simulink model "hopper_6dof"  (R2026b)
settings: Solver=FixedStepAuto  StopTime=tgrid(end)  FixedStep=1e-3  RelTol=1e-5
undefined symbols (not defined in the file): cg_init, controller_start_time, fdir_params, fsw_latency, fsw_period, g, IN, K1flat, K1flat_lo, K2grid, Klqi, nav_dt, nav_g, nav_init, nav_Qc, nav_reset, OUT, p, sensor_params, Target_Trajectory, tgrid, u_hold_command, unom, VEH
libraries: fl_lib x43, nesl_utility x31, SimscapeFluids_lib x13, slpidlib x3, simulink_extras x2, commrandsrc3 x1, dspsrcs4 x1, matrix_library x1, aerolibutil x1
(part 5 of 6)

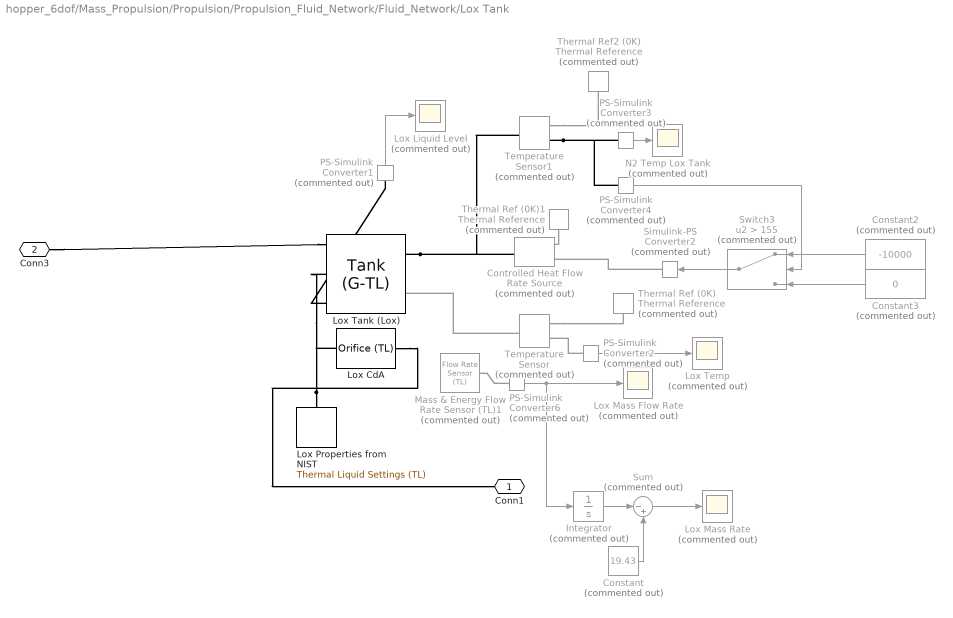
== system hopper_6dof/Mass_Propulsion/Propulsion/Propulsion_Fluid_Network/Fluid_Network/Lox Tank ==
  Constant : Constant  Commented=on  Value=19.43
  Constant2 : Constant  Commented=on  Value=-10000
  Constant3 : Constant  Commented=on  Value=0
  Controlled Heat Flow Rate Source : fl_lib/Thermal/Thermal Sources/Controlled Heat Flow Rate Source  Commented=on
  Integrator : Integrator  Commented=on
  Lox CdA : SimscapeFluids_lib/Thermal Liquid/Valves & Orifices/Orifice (TL)  orifice_type=foundation.enum.constant_variable.constant  constant_orifice_spec=fluids.thermal_liquid.valves.enum.ConstantOrificeSpec.Area  variable_orifice_spec=fluids.thermal_liquid.valves.enum.orifice_spec.linear  orifice_area_constant=100 mm^2  p_diff_TLU_constant=[-4, -3, -2, -1, -.5, 0, .5, 1, 2, 3, 4] MPa  vol_flow_TLU_constant=[-2.44, -2.12, -1.68, -1.22, -.84, 0, .85, 1.21, 1.7, 2.09, 2.41] .* 1e-3 m^3/s  mdot_TLU_constant=[-2.44, -2.12, -1.68, -1.22, -.84, 0, .85, 1.21, 1.7, 2.09, 2.41] kg/s  S_min=0 m  del_S=5e-3 m  open_orientation=fluids.thermal_liquid.valves.enum.orifice_orientation.positive  area_max=1e-4 m^2  area_leak=1e-10 m^2  S_TLU=[0, .002, .004, .007, .017] m  orifice_area_TLU=[1e-09, 2.0352e-07, 4.0736e-05, .00011438, .00034356] m^2  Cd=1  Re_c=150  smoothing_factor=0.01  pressure_recovery=simscape.enum.onoff.off  S_flow_TLU=[0, .002, .004, .007, .017] m  p_diff_TLU=[.3, .5, .7] MPa  vol_flow_TLU=1e-3 * [1.7e-05, 2e-05, 2.6e-05; .0035, .0045, .0053; .7, .9, 1.06; 1.96, 2.5, 3; 6, 7.7, 9.13] m^3/s  mdot_TLU=[1.7e-05, 2e-05, 2.6e-05; .0035, .0045, .0053; .7, .9, 1.06; 1.96, 2.5, 3; 6, 7.7, 9.13] kg/s  T_ref_in=293.15 K  p_ref_in=0.101325 MPa  area=0.01 m^2
  Lox Liquid Level : Scope  Commented=on
      settings: ActiveDisplayYMinimum=0.2716109686745361  ActiveDisplayYMaximum=0.57353060563413627  DataLoggingVariableName=ScopeData8
  Lox Mass Flow Rate : Scope  Commented=on
      settings: ActiveDisplayYMinimum=-0.047859120665806151  ActiveDisplayYMaximum=0.43156982443661435  DataLoggingVariableName=ScopeData9
  Lox Mass Rate : Scope  Commented=on
      settings: ActiveDisplayYMinimum=1.5375974928550786  ActiveDisplayYMaximum=10.60693361190499  DataLoggingVariableName=ScopeData19
  Lox Properties from NIST : fl_lib/Thermal Liquid/Utilities/Thermal Liquid Settings (TL)  table_dimensions=foundation.enum.table_dimensions_TL.two_dimensional  T_TLU=[70 : 10 : 130]' K  p_TLU=[10:10:600] psi  T_atm=100 K  p_atm=0.101325 MPa  pT_region_flag=foundation.enum.pT_region_TL.min_max  T_min=70 K  T_max=130 K  p_min=10 psi  p_max=600 psi  T_min_1D=273.16 K  T_max_1D=363.16 K  p_min_1D=0.05 MPa  p_max_1D=50 MPa  pT_validity_TLU=[1, 1, 1, 1, 1, 1, 1, 1, 1, 1, 1, 1; 1, 1, 1, 1, 1, 1, 1, 1, 1, 1, 1, 1; 1, 1, 1, 1, 1, 1, 1, 1, 1, 1, 1, 1; 1, 1, 1, 1, 1, 1, 1, 1, 1, 1, 1, 1; 1, 1, 1, 1, 1, 1, 1, 1, 1, 1, 1, 1; 0, 1, 1, 1, 1, 1, 1, 1, 1, 1, 1, 1; 0, 1, 1, 1, 1, 1, 1, 1, 1, 1, 1, 1; 0, 1, 1, 1, 1, 1, 1, 1, 1, 1, 1, 1; 0, 1, 1, 1, 1, 1, 1, 1, 1, 1, 1, 1; 0, 1, 1, 1, 1, 1, 1, 1, 1, 1, 1, 1; 0, 0, 1, 1, 1, 1, 1, 1, 1, 1, 1, 1]  properties_range_check=simscape.enum.assert.action.error  rho_parameterization_2D=foundation.enum.rho_parameterization_2D.rho_table  rho_parameterization_1D=foundation.enum.rho_parameterization_1D.rho_vector  rho_TLU=[1237,1190.5,1142.1,1141,1141,1141,1141] kg/m^3  beta_TLU=[1.9649, 1.9654, 1.9929, 2.0213, 2.0499, 2.0787, 2.1078, 2.1372, 2.1668, 2.1966, 2.2268, 2.2572; 2.0913, 2.0918, 2.1191, 2.1471, 2.1752, 2.2036, 2.2322, 2.261, 2.2899, 2.3191, 2.3485, 2.3781; 2.1786, 2.1791, 2.2067, 2.235, 2.2634, 2.2919, 2.3206, 2.3494, 2.3784, 2.4075, 2.4367, 2.4661; 2.2332, 2.2337, 2.2619, 2.2908, 2.3197, 2.3487, 2.3778, 2.407, 2.4363, 2.4657, 2.4951, 2.5246; 2.26, 2.2605, 2.2895, 2.3191, 2.3487, 2.3784, 2.4081, 2.4378, 2.4675, 2.4973, 2.5272, 2.5571; 2.2638, 2.2638, 2.2936, 2.324, 2.3544, 2.3848, 2.4151, 2.4455, 2.4758, 2.5062, 2.5365, 2.5669; 2.2472, 2.2472, 2.2779, 2.3092, 2.3403, 2.3715, 2.4025, 2.4336, 2.4646, 2.4955, 2.5264, 2.5573; 2.214, 2.214, 2.2455, 2.2776, 2.3096, 2.3415, 2.3733, 2.405, 2.4367, 2.4683, 2.4998, 2.5313; 2.1668, 2.1668, 2.1992, 2.2321, 2.2649, 2.2976, 2.3301, 2.3626, 2.3949, 2.4272, 2.4593, 2.4914; 2.1081, 2.1081, 2.1413, 2.175, 2.2086, 2.2421, 2.2754, 2.3085, 2.3415, 2.3744, 2.4072, 2.4399; 2.0494, 2.0494, 2.0739, 2.1084, 2.1428, 2.177, 2.211, 2.2449, 2.2786, 2.3121, 2.3455, 2.3788] GPa  alpha_TLU=1e-4 * [-.679, -.676, -.49, -.307, -.13, .041, .206, .365, .519, .668, .811, .949; .878, .881, .998, 1.114, 1.227, 1.337, 1.445, 1.549, 1.651, 1.75, 1.846, 1.939; 2.068, 2.069, 2.141, 2.213, 2.283, 2.352, 2.42, 2.486, 2.551, 2.614, 2.676, 2.736; 3.034, 3.035, 3.074, 3.113, 3.152, 3.191, 3.229, 3.267, 3.305, 3.341, 3.377, 3.413; 3.855, 3.856, 3.87, 3.884, 3.899, 3.914, 3.93, 3.946, 3.961, 3.977, 3.993, 4.009; 4.578, 4.578, 4.572, 4.566, 4.562, 4.558, 4.555, 4.552, 4.55, 4.549, 4.548, 4.547; 5.233, 5.233, 5.209, 5.186, 5.165, 5.144, 5.125, 5.107, 5.09, 5.074, 5.059, 5.045; 5.84, 5.84, 5.801, 5.762, 5.725, 5.691, 5.657, 5.625, 5.595, 5.566, 5.538, 5.512; 6.414, 6.414, 6.36, 6.307, 6.256, 6.208, 6.161, 6.117, 6.074, 6.033, 5.994, 5.956; 6.967, 6.967, 6.898, 6.831, 6.766, 6.705, 6.646, 6.589, 6.535, 6.482, 6.432, 6.384; 7.519, 7.519, 7.423, 7.342, 7.264, 7.189, 7.118, 7.049, 6.983, 6.92, 6.859, 6.8] 1/K  rho_TLU_2=|  rho_ref_3=998.21 kg/m^3  T_ref_3=293.16 K  p_ref_3=0.101325 MPa  beta_const_3=2.1791 GPa  alpha_const_3=2.0691e-4 1/K  rho_TLU_4=[999.84; 999.7; 998.2; 995.65; 992.21; 988.03; 983.19; 977.76; 971.78; 965.3; 958.8] kg/m^3  beta_const_4=2.1791 GPa  p_ref_4=0.101325 MPa  rho_ref_5=998.21 kg/m^3  T_ref_5=293.16 K  p_ref_5=0.101325 MPa  beta_const_5=2.1791 GPa  alpha_const_5=2.0691e-4 1/K  u_parameterization_2D=foundation.enum.u_parameterization_2D.u_cp  u_parameterization_1D=foundation.enum.u_parameterization_1D.u  u_TLU=|  cp_TLU=|  u_TLU_2=[.0002, .0018, .086, .1588, .219, .267, .3034, .3288, .3436, .3483, .3435, .3294; 42.062, 42.06, 41.935, 41.804, 41.668, 41.527, 41.382, 41.233, 41.081, 40.924, 40.763, 40.599; 83.953, 83.948, 83.651, 83.349, 83.049, 82.749, 82.451, 82.153, 81.856, 81.56, 81.265, 80.971; 125.77, 125.76, 125.31, 124.86, 124.41, 123.97, 123.53, 123.1, 122.68, 122.25, 121.84, 121.42; 167.57, 167.56, 166.96, 166.37, 165.79, 165.21, 164.65, 164.09, 163.54, 163, 162.46, 161.94; 209.36, 209.36, 208.63, 207.9, 207.19, 206.48, 205.79, 205.11, 204.45, 203.79, 203.14, 202.5; 251.19, 251.19, 250.33, 249.47, 248.62, 247.79, 246.98, 246.18, 245.39, 244.62, 243.86, 243.12; 293.06, 293.06, 292.07, 291.07, 290.1, 289.14, 288.2, 287.28, 286.38, 285.49, 284.62, 283.77; 334.99, 334.99, 333.86, 332.73, 331.63, 330.54, 329.48, 328.44, 327.41, 326.41, 325.43, 324.46; 377, 377, 375.73, 374.46, 373.22, 372, 370.81, 369.64, 368.5, 367.38, 366.27, 365.19; 419.01, 419.01, 417.69, 416.27, 414.89, 413.54, 412.21, 410.91, 409.64, 408.4, 407.17, 405.98] kJ/kg  cp_TLU_3=[4.2199, 4.2194, 4.1957, 4.1726, 4.1508, 4.13, 4.1103, 4.0916, 4.0738, 4.0569, 4.0408, 4.0254; 4.1955, 4.1951, 4.1769, 4.1592, 4.1422, 4.1259, 4.1103, 4.0954, 4.0812, 4.0676, 4.0545, 4.0421; 4.1843, 4.184, 4.169, 4.1543, 4.1401, 4.1264, 4.1133, 4.1007, 4.0885, 4.0768, 4.0656, 4.0548; 4.1801, 4.1798, 4.1667, 4.1538, 4.1413, 4.1293, 4.1177, 4.1064, 4.0956, 4.0851, 4.075, 4.0653; 4.1796, 4.1794, 4.1675, 4.1558, 4.1444, 4.1334, 4.1227, 4.1123, 4.1023, 4.0926, 4.0832, 4.0741; 4.1813, 4.1813, 4.1702, 4.1592, 4.1484, 4.138, 4.1279, 4.1181, 4.1086, 4.0993, 4.0903, 4.0816; 4.185, 4.185, 4.1742, 4.1636, 4.1532, 4.1432, 4.1334, 4.1239, 4.1146, 4.1056, 4.0969, 4.0884; 4.1901, 4.1901, 4.1795, 4.169, 4.1588, 4.1489, 4.1393, 4.1299, 4.1207, 4.1118, 4.1032, 4.0947; 4.1968, 4.1968, 4.1862, 4.1757, 4.1655, 4.1555, 4.1458, 4.1364, 4.1273, 4.1183, 4.1096, 4.1012; 4.2052, 4.2052, 4.1944, 4.1837, 4.1733, 4.1632, 4.1534, 4.1438, 4.1345, 4.1255, 4.1166, 4.108; 4.2136, 4.2136, 4.2045, 4.1935, 4.1828, 4.1724, 4.1623, 4.1524, 4.1429, 4.1335, 4.1245, 4.1157] kJ/(K*kg)  u_TLU_4=[.0018; 42.06; 83.948; 125.76; 167.56; 209.36; 251.19; 293.06; 334.99; 377; 418.01] kJ/kg  cp_TLU_5=[4.2199; 4.1955; 4.1843; 4.1801; 4.1796; 4.1813; 4.185; 4.1901; 4.1968; 4.2052; 4.2136] kJ/(K*kg)  nu_TLU=|  nu_TLU_2=[1.7917; 1.3061; 1.0032; .8006; .6577; .553; .4739; .4127; .3643; .3254; .2866] mm^2/s  k_TLU=|  k_TLU_2=[561.04; 580.02; 598.44; 615.48; 630.6; 643.61; 654.39; 663.13; 670.02; 675.27; 680.52] mW/(K*m)  air_fraction=0  R_air=0.287 kJ/(K*kg)  air_dissolution_model=false  p_crit=3 MPa
      rho_TLU_2=|
      | [1237.088,1237.184,1237.28,1237.376,1237.504,1237.6,1237.696,1237.792,1237.888,1237.984,1238.08,1238.176,1238.272,1238.4,1238.496,1238.592,1238.688,1238.784,1238.88,1238.976,1239.072,1239.168,1239.264,1239.392,1239.488,1239.584,1239.68,1239.776,1239.872,1239.968,1240.064,1240.16,1240.256,1240.352,1240.448,1240.544,1240.64,1240.768,1240.864,1240.96,1241.056,1241.152,1241.248,1241.344,1241.44,1241.536,1241.632,1241.728,1241.824,1241.92,1242.0,1242.1,1242.2,1242.3,1242.4,1242.5,1242.6,1242.7,1242.71,1242.8;
      | 
      | 1190.56,1190.688,1190.816,1190.944,1191.072,1191.2,1191.296,1191.424,1191.552,1191.68,1191.808,1191.904,1192.032,1192.16,1192.288,1192.416,1192.512,1192.64,1192.768,1192.896,1192.992,1193.12,1193.248,1193.376,1193.504,1193.6,1193.728,1193.856,1193.984,1194.08,1194.208,1194.336,1194.464,1194.56,1194.688,1194.816,1194.912,1195.04,1195.168,1195.296,1195.392,1195.52,1195.648,1195.744,1195.872,1196,1196.128,1196.224,1196.352,1196.48,1196.5,1196.7,1196.8,1196.9,1197.0,1197.1,1197.2,1197.4,1197.5,1197.6;
      | 
      | 3.013,1142.24,1142.4,1142.528,1142.688,1142.848,1143.008,1143.136,1143.296,1143.456,1143.616,1143.744,1143.904,1144.064,1144.224,1144.352,1144.512,1144.672,1144.832,1144.96,1145.12,1145.28,1145.408,1145.568,1145.728,1145.856,1146.016,1146.176,1146.304,1146.464,1146.624,1146.752,1146.912,1147.072,1147.2,1147.36,1147.488,1147.648,1147.808,1147.936,1148.096,1148.256,1148.384,1148.544,1148.672,1148.832,1148.96,1149.12,1149.28,1149.408,1149.5,1149.7,1149.8,1150.0,1150.1,1150.2,1150.4,1150.5,1150.7,1150.8;
      | 
      | 2.697,5.487,8.38,1090.976,1091.2,1091.392,1091.584,1091.776,1091.968,1092.16,1092.384,1092.576,1092.768,1092.96,1093.152,1093.344,1093.536,1093.728,1093.92,1094.112,1094.304,1094.496,1094.688,1094.88,1095.072,1095.264,1095.456,1095.648,1095.84,1096.032,1096.224,1096.416,1096.608,1096.8,1096.992,1097.184,1097.376,1097.536,1097.728,1097.92,1098.112,1098.304,1098.496,1098.688,1098.848,1099.04,1099.232,1099.424,1099.616,1099.776,1099.9,1100.1,1100.3,1100.5,1100.7,1100.9,1101.0,1101.2,1101.4,1101.6;
      | 
      | 2.442,4.948,7.521,10.167,12.894,15.709,18.623,1035.552,1035.808,1036.064,1036.352,1036.608,1036.864,1037.12,1037.408,1037.664,1037.92,1038.176,1038.432,1038.688,1038.944,1039.2,1039.488,1039.744,1040,1040.256,1040.512,1040.768,1041.024,1041.248,1041.504,1041.76,1042.016,1042.272,1042.528,1042.784,1043.04,1043.264,1043.52,1043.776,1044.032,1044.256,1044.512,1044.768,1045.024,1045.248,1045.504,1045.76,1045.984,1046.24,1046.4,1046.7,1046.9,1047.2,1047.4,1047.6,1047.9,1048.1,1048.4,1048.6;
      | 
      | 2.233,4.51,6.834,9.207,11.634,14.116,16.659,19.267,21.944,24.697,27.532,30.458,33.485,36.621,973.952,974.336,974.72,975.104,975.488,975.84,976.224,976.608,976.96,977.344,977.728,978.08,978.464,978.816,979.168,979.552,979.904,980.256,980.64,980.992,981.344,981.696,982.048,982.4,982.752,983.104,983.456,983.808,984.16,984.512,984.864,985.216,985.536,985.888,986.24,986.56,986.87,987.21,987.55,987.89,988.22,988.56,988.89,989.22,989.55,989.88;
      | 
      | 2.057,4.146,6.268,8.426,10.62,12.852,15.125,17.441,19.801,22.209,24.666,27.176,29.743,32.368,35.059,37.818,40.653,43.565,46.563,49.658,52.858,56.17,59.61,63.197,66.944,902.912,903.52,904.128,904.704,905.312,905.92,906.496,907.104,907.68,908.256,908.832,909.408,909.952,910.528,911.104,911.648,912.224,912.768,913.312,913.856,914.4,914.944,915.488,916,916.544,917.03,917.56,918.08,918.6,919.12,919.63,920.14,920.65,921.16,921.66] kg/m^3
      u_TLU=|
      | [-167.43125,-167.44375,-167.459375,-167.475,-167.4875,-167.503125,-167.515625,-167.53125,-167.546875,-167.559375,-167.575,-167.5875,-167.603125,-167.615625,-167.63125,-167.646875,-167.659375,-167.675,-167.6875,-167.703125,-167.715625,-167.73125,-167.74375,-167.759375,-167.771875,-167.7875,-167.8,-167.815625,-167.828125,-167.84375,-167.85625,-167.871875,-167.884375,-167.9,-167.9125,-167.928125,-167.940625,-167.95625,-167.96875,-167.984375,-167.996875,-168.0125,-168.025,-168.040625,-168.053125,-168.06875,-168.08125,-168.09375,-168.109375,-168.121875,-168.14,-168.16,-168.17,-168.18,-168.20,-168.21,-168.23,-168.24,-168.25,-168.27;
      | -150.64375,-150.6625,-150.68125,-150.696875,-150.715625,-150.734375,-150.753125,-150.771875,-150.790625,-150.809375,-150.825,-150.84375,-150.8625,-150.88125,-150.9,-150.91875,-150.934375,-150.953125,-150.971875,-150.990625,-151.00625,-151.025,-151.04375,-151.0625,-151.078125,-151.096875,-151.115625,-151.134375,-151.15,-151.16875,-151.1875,-151.20625,-151.221875,-151.240625,-151.259375,-151.275,-151.29375,-151.3125,-151.328125,-151.346875,-151.365625,-151.38125,-151.4,-151.41875,-151.434375,-151.453125,-151.46875,-151.4875,-151.50625,-151.521875,-151.55,-151.56,-151.58,-151.60,-151.62,-151.63,-151.65,-151.67,-151.68,-151.70;
      | 57.3375,-133.784375,-133.80625,-133.83125,-133.853125,-133.878125,-133.9,-133.925,-133.946875,-133.971875,-133.99375,-134.01875,-134.040625,-134.065625,-134.0875,-134.1125,-134.134375,-134.159375,-134.18125,-134.203125,-134.228125,-134.25,-134.271875,-134.296875,-134.31875,-134.34375,-134.365625,-134.3875,-134.4125,-134.434375,-134.45625,-134.478125,-134.503125,-134.525,-134.546875,-134.56875,-134.59375,-134.615625,-134.6375,-134.659375,-134.684375,-134.70625,-134.728125,-134.75,-134.771875,-134.79375,-134.81875,-134.840625,-134.8625,-134.884375,-134.91,-134.93,-134.96,-134.98,-135.00,-135.02,-135.04,-135.07,-135.09,-135.11;
      | 63.946875,63.184375,62.378125,-116.6875,-116.71875,-116.75,-116.78125,-116.8125,-116.84375,-116.871875,-116.903125,-116.934375,-116.965625,-116.996875,-117.025,-117.05625,-117.0875,-117.11875,-117.146875,-117.178125,-117.209375,-117.2375,-117.26875,-117.296875,-117.328125,-117.359375,-117.3875,-117.41875,-117.446875,-117.478125,-117.50625,-117.5375,-117.565625,-117.596875,-117.625,-117.653125,-117.684375,-117.7125,-117.74375,-117.771875,-117.8,-117.83125,-117.859375,-117.8875,-117.915625,-117.946875,-117.975,-118.003125,-118.03125,-118.0625,-118.09,-118.12,-118.15,-118.18,-118.21,-118.24,-118.27,-118.29,-118.32,-118.35;
      | 70.5375,69.884375,69.209375,68.515625,67.796875,67.046875,66.25625,-99.165625,-99.209375,-99.25,-99.29375,-99.334375,-99.375,-99.415625,-99.459375,-99.5,-99.540625,-99.58125,-99.621875,-99.6625,-99.703125,-99.74375,-99.784375,-99.825,-99.865625,-99.90625,-99.946875,-99.9875,-100.028125,-100.065625,-100.10625,-100.146875,-100.184375,-100.225,-100.265625,-100.303125,-100.34375,-100.38125,-100.421875,-100.459375,-100.5,-100.5375,-100.578125,-100.615625,-100.653125,-100.69375,-100.73125,-100.76875,-100.809375,-100.846875,-100.89,-100.93,-110.96,-101.00,-101.04,-101.08,-101.11,-101.15,-101.19,-101.23;
      | 77.11875,76.55625,75.978125,75.390625,74.7875,74.16875,73.5375,72.8875,72.215625,71.525,70.809375,70.0625,69.28125,68.459375,-80.9625,-81.021875,-81.08125,-81.140625,-81.2,-81.25625,-81.315625,-81.375,-81.43125,-81.490625,-81.546875,-81.60625,-81.6625,-81.71875,-81.778125,-81.834375,-81.890625,-81.946875,-82.003125,-82.059375,-82.115625,-82.16875,-82.225,-82.28125,-82.334375,-82.390625,-82.446875,-82.5,-82.553125,-82.609375,-82.6625,-82.715625,-82.76875,-82.821875,-82.878125,-82.93125,-82.986,-83.039,-83.091,-83.144,-83.196,-83.248,-83.300,-83.352,-83.404,-83.455;
      | 83.6875,83.2,82.7,82.19375,81.68125,81.15625,80.621875,80.078125,79.525,78.959375,78.38125,77.790625,77.1875,76.56875,75.9375,75.284375,74.6125,73.921875,73.209375,72.46875,71.7,70.896875,70.05625,69.175,68.240625,-61.65625,-61.75,-61.840625,-61.934375,-62.025,-62.115625,-62.203125,-62.29375,-62.38125,-62.471875,-62.559375,-62.646875,-62.73125,-62.81875,-62.903125,-62.9875,-63.075,-63.159375,-63.240625,-63.325,-63.40625,-63.490625,-63.571875,-63.653125,-63.734375,-63.818,-63.898,-63.978,-64.057,-64.136,-64.215,-64.293,-64.371,-64.449,-64.526] kJ/kg
      cp_TLU=|
      | [1.67790625,1.67775,1.67759375,1.67746875,1.6773125,1.67715625,1.677,1.676875,1.67671875,1.6765625,1.6764375,1.67628125,1.67615625,1.676,1.67584375,1.67571875,1.6755625,1.6754375,1.67528125,1.675125,1.675,1.67484375,1.67471875,1.6745625,1.6744375,1.67428125,1.67415625,1.674,1.673875,1.67371875,1.67359375,1.6734375,1.6733125,1.67315625,1.67303125,1.67290625,1.67275,1.672625,1.67246875,1.67234375,1.67221875,1.6720625,1.6719375,1.6718125,1.67165625,1.67153125,1.67140625,1.67125,1.671125,1.671,1.6709,1.6708,1.6707,1.6705,1.6704,1.6703,1.6701,1.67,1.6699,1.6697;
      | 1.681375,1.68115625,1.6809375,1.68071875,1.6805,1.68028125,1.6800625,1.67984375,1.679625,1.67940625,1.6791875,1.67896875,1.67875,1.6785625,1.67834375,1.678125,1.67790625,1.6776875,1.67746875,1.67728125,1.6770625,1.67684375,1.676625,1.6764375,1.67621875,1.676,1.67578125,1.67559375,1.675375,1.6751875,1.67496875,1.67475,1.6745625,1.67434375,1.67415625,1.6739375,1.67375,1.67353125,1.67334375,1.673125,1.6729375,1.67271875,1.67253125,1.6723125,1.672125,1.6719375,1.67171875,1.67153125,1.6713125,1.671125,1.671,1.6708,1.6706,1.6704,1.6702,1.67,1.6698,1.6696,1.6694,1.6692;
      | 0.93946875,1.69859375,1.69825,1.697875,1.69753125,1.6971875,1.69684375,1.69646875,1.696125,1.69578125,1.6954375,1.69509375,1.69475,1.69440625,1.6940625,1.69371875,1.693375,1.69303125,1.69271875,1.692375,1.69203125,1.6916875,1.691375,1.69103125,1.6906875,1.690375,1.69003125,1.68971875,1.689375,1.6890625,1.68871875,1.68840625,1.6880625,1.68775,1.6874375,1.68709375,1.68678125,1.68646875,1.68615625,1.68584375,1.6855,1.6851875,1.684875,1.6845625,1.68425,1.6839375,1.683625,1.6833125,1.683,1.6826875,1.6825,1.6821,1.6818,1.6815,1.6812,1.6809,1.6806,1.6803,1.68,1.6797;
      | 0.92621875,0.947625,0.97703125,1.73728125,1.7366875,1.73609375,1.73553125,1.7349375,1.734375,1.73378125,1.73321875,1.73265625,1.73209375,1.7315,1.7309375,1.730375,1.72984375,1.72928125,1.72871875,1.72815625,1.727625,1.7270625,1.72653125,1.72596875,1.7254375,1.724875,1.72434375,1.7238125,1.72328125,1.72275,1.72221875,1.7216875,1.72115625,1.720625,1.720125,1.71959375,1.7190625,1.7185625,1.71803125,1.71753125,1.71703125,1.7165,1.716,1.7155,1.715,1.7145,1.714,1.7135,1.713,1.7125,1.7121,1.7116,1.7111,1.7106,1.7101,1.7096,1.7092,1.7087,1.7082,1.7077;
      | 0.9244375,0.94053125,0.95809375,0.9775625,0.99996875,1.027,1.06146875,1.806625,1.80559375,1.8045625,1.8035625,1.80253125,1.80153125,1.80053125,1.79953125,1.79853125,1.7975625,1.7965625,1.79559375,1.794625,1.79365625,1.7926875,1.79175,1.79078125,1.78984375,1.78890625,1.78796875,1.78703125,1.786125,1.7851875,1.78428125,1.783375,1.78246875,1.7815625,1.78065625,1.77978125,1.778875,1.778,1.777125,1.77625,1.775375,1.7745,1.77365625,1.77278125,1.7719375,1.77109375,1.77025,1.76940625,1.7685625,1.76771875,1.767,1.7661,1.7653,1.7645,1.7637,1.7629,1.7621,1.7613,1.7605,1.7597;
      | 0.922125,0.93528125,0.9491875,0.96396875,0.97971875,0.9965625,1.01475,1.03465625,1.05665625,1.081375,1.10965625,1.14259375,1.18165625,1.2289375,1.92671875,1.9246875,1.9226875,1.9206875,1.91871875,1.91675,1.9148125,1.912875,1.91096875,1.9090625,1.9071875,1.9053125,1.90346875,1.901625,1.8998125,1.898,1.89621875,1.8944375,1.8926875,1.8909375,1.8891875,1.88746875,1.88575,1.8840625,1.882375,1.88071875,1.8790625,1.87740625,1.87578125,1.87415625,1.87253125,1.8709375,1.869375,1.86778125,1.86621875,1.8646875,1.8632,1.8617,1.8602,1.8587,1.8572,1.8557,1.8542,1.8527,1.8513,1.8498;
      | 0.919875,0.9304375,0.9415,0.95309375,0.96521875,0.9779375,0.99128125,1.00534375,1.0201875,1.03590625,1.0525625,1.070375,1.0894375,1.10996875,1.1321875,1.156375,1.1829375,1.21228125,1.2449375,1.281625,1.32321875,1.370875,1.4260625,1.49084375,1.5679375,2.15015625,2.14528125,2.1404375,2.13571875,2.13103125,2.1264375,2.12190625,2.1174375,2.11303125,2.1086875,2.10440625,2.10015625,2.096,2.09190625,2.08784375,2.08384375,2.07990625,2.07603125,2.0721875,2.06840625,2.06465625,2.06096875,2.0573125,2.05371875,2.05015625,2.0467,2.0433,2.0398,2.0365,2.0331,2.0298,2.0265,2.0233,2.0201,2.017] kJ/(K*kg)
      nu_TLU=|
      | [0.300698091000802,0.300852581346024,0.301007047717574,0.30116149012103,0.301308116983864,0.301462508080155,0.301616875226227,0.301771218427652,0.301925537690001,0.302079833018844,0.302234104419747,0.302388351898276,0.302542575459996,0.302688953488372,0.302843125855877,0.302997274324394,0.303151398899481,0.303305499586691,0.303459576391579,0.303613629319696,0.303767658376592,0.303921663567813,0.304075644898908,0.304221747437453,0.304375677699179,0.304529584118543,0.304683466701084,0.30483732545234,0.304991160377845,0.305144971483135,0.305298758773741,0.305452522255193,0.30560626193302,0.30575997781275,0.305913669899907,0.306067338200015,0.306220982718597,0.306366701913653,0.306528354436908,0.306681923671996,0.306835469148854,0.306988990872995,0.307142488849932,0.307295963085172,0.307449413584225,0.307602840352595,0.307756243395789,0.307909622719307,0.308062978328652,0.308216310229322,0.3083,0.3084,0.3086,0.3088,0.3089,0.3091,0.3093,0.3094,0.3096,0.3098;
      | 0.219484948259643,0.21960412803354,0.219714884583345,0.219834014025848,0.219944722065501,0.220063801208865,0.220188769205974,0.220299406424581,0.220418412289183,0.220529001074114,0.220647956717861,0.220764423980455,0.220883331991088,0.221002214467857,0.221112684183687,0.221231516517725,0.221347877421779,0.221466662194795,0.221585421473413,0.221695772305381,0.221820431318902,0.221930736221,0.222049397945775,0.222159654626874,0.2222782663485,0.222402815013405,0.222513001286725,0.222631540152246,0.222741678280446,0.222866139622136,0.222976231946194,0.223094673525708,0.223213089720578,0.223329091883204,0.223447460759629,0.223557434784938,0.223681743927586,0.22379167224528,0.22390994404134,0.224028190506787,0.224144046471785,0.224262245717345,0.224372055989723,0.224496213236278,0.224614339996254,0.224724080267559,0.224842157361085,0.224957867422824,0.225075897394747,0.225185544263172,0.2253,0.2254,0.2255,0.2256,0.2257,0.2258,0.2259,0.2260,0.2261,0.2262;
      | 2.3012413456229,0.171347527664939,0.171446078431373,0.171540653708268,0.171639152594584,0.171737623900991,0.171836067639072,0.171930548946057,0.1720289408867,0.172127305292027,0.172216897979741,0.172320029656986,0.172418314823622,0.172507831729693,0.172606063148474,0.172709096501776,0.172798537717385,0.172896690056191,0.17299481495975,0.173089016210173,0.173187089562666,0.173285135512713,0.173379267474996,0.173477261934691,0.17357522902469,0.173669291778374,0.17376720743864,0.173865095761907,0.173959089386411,0.174056926340469,0.174146014735432,0.174248660564795,0.174346418905723,0.174435432126318,0.174538005578801,0.174635685399526,0.174729496081876,0.174827124693286,0.174916013828097,0.175018467928526,0.175116018172696,0.175204832371875,0.175307214311589,0.175404686281065,0.17549831457544,0.175595735494833,0.175689319036346,0.175786688944584,0.175884031741612,0.175977546702302,0.1761,0.1762,0.1763,0.1764,0.1765,0.1766,0.1767,0.1768,0.1769,0.1770;
      | 2.85843745179701,1.40626822582527,0.921651836859391,0.139865588243921,0.139956011730205,0.140041341699408,0.140126641651032,0.140221070988921,0.140306309342398,0.14039151772634,0.140481735360459,0.140566880473303,0.140651995666052,0.140737080954472,0.140831284212991,0.140916308133579,0.141001302197641,0.14109540946195,0.141180342255375,0.141265245239975,0.141350118431441,0.141444098470894,0.141528910520623,0.141613692824784,0.141698445399024,0.141783168258977,0.141876990038851,0.141961651917404,0.14204628412907,0.14213088668944,0.142215459614093,0.142309123544348,0.142393635647378,0.142478118161926,0.142562571103527,0.142646994487707,0.14273138832998,0.142819916613214,0.142913362873134,0.142997668318275,0.14308194428255,0.143166190781423,0.143250407830343,0.143334595444749,0.143422930195987,0.143507060707527,0.143600259089983,0.14368432924877,0.143768370049181,0.143856567155493,0.1439,0.1440,0.1441,0.1442,0.1443,0.1444,0.1445,0.1446,0.1447,0.1448;
      | 3.46737713402251,1.71372728154712,1.12873888439774,0.836008560727662,0.660077242834098,0.542540026888291,0.458327247577153,0.117367355767745,0.117454200006179,0.117541001328103,0.117624127709504,0.117710841513861,0.117797512499228,0.11787449861154,0.117957447792961,0.118043991118512,0.118130491752736,0.118216949727214,0.118303365073495,0.1183897378231,0.118476068007515,0.118562355658199,0.118635328161556,0.118721531453896,0.118807692307692,0.118893810754276,0.118979886824948,0.119065920550978,0.119142306037133,0.119231921693967,0.11931783267275,0.119403701428352,0.119479931210269,0.119565717969973,0.119651462598606,0.119727575413508,0.119813238226722,0.119902536654193,0.119978534191966,0.120064075050586,0.120149573959419,0.120229139214905,0.120314558377501,0.1203999356795,0.120475701993447,0.1205646889542,0.120640380142018,0.120725596695226,0.120814467525316,0.120890044349289,0.1209,0.1210,0.1211,0.1212,0.1213,0.1214,0.1215,0.1216,0.1217,0.1218;
      | 4.1267001805882,2.04580731568864,1.35196675251698,1.00487235854303,0.7964258698941,0.657316838191957,0.557841913177103,0.483103647295255,0.424857092860476,0.378142856217365,0.33980229895745,0.307732767043843,0.280461582568807,0.256971447920308,0.10005421211723,0.100145124474514,0.100234939264609,0.100324683315831,0.100414356711718,0.100506230529595,0.100595764906415,0.100684204921524,0.100775876187357,0.100863155654509,0.100950366564116,0.101041837068542,0.101127890244301,0.101218206486204,0.101308457792738,0.101394310868642,0.101483410619816,0.101571426239676,0.1016570810899,0.101744968358559,0.101833811589004,0.101925647043484,0.102011306982958,0.102096905537459,0.102182442772948,0.102267918755289,0.102353333550255,0.102438687223523,0.102523979840676,0.102609211467204,0.102694382168502,0.102779492009874,0.102867881031236,0.102952870914343,0.103037800129786,0.103126013623094,0.1032,0.1033,0.1034,0.1035,0.1036,0.1037,0.1038,0.1039,0.1040,0.1041;
      | 4.83498179753255,2.40209651898734,1.59107297835409,1.18538739080896,0.941822099014675,0.779460462105368,0.663319546406584,0.576172412527751,0.508300473504743,0.453967464914556,0.409426000882177,0.372272625579917,0.34075198769191,0.313704893722195,0.29016634720701,0.269557031646641,0.251274204974811,0.234983289261055,0.220367156896433,0.207118346436396,0.19507128586996,0.184049735088019,0.173931715696801,0.164549470859284,0.155831739961759,0.0860150269350723,0.0861198423941916,0.0862234108444822,0.0863298935342388,0.0864320808737761,0.0865341310490993,0.0866379995057893,0.0867375736409497,0.0868400757976379,0.0869413469330233,0.0870424897010669,0.0871424047292304,0.0872452612885075,0.0873438268784705,0.0874422678420905,0.0875425602864263,0.0876385624583436,0.0877386148506521,0.0878363582215059,0.0879339852230548,0.0880314960629921,0.0881288909485171,0.0882239854591212,0.0883231441048035,0.0884180137560226,0.0885,0.0886,0.0887,0.0888,0.0889,0.0890,0.0891,0.0892,0.0893,0.0894] mm^2/s
      k_TLU=|
      | [0.17977,0.1798,0.17984,0.17987,0.17991,0.17994,0.17998,0.18001,0.18005,0.18008,0.18012,0.18015,0.18019,0.18022,0.18026,0.18029,0.18033,0.18037,0.1804,0.18044,0.18047,0.18051,0.18054,0.18058,0.18061,0.18065,0.18068,0.18072,0.18075,0.18079,0.18082,0.18086,0.18089,0.18093,0.18096,0.181,0.18103,0.18107,0.1811,0.18113,0.18117,0.1812,0.18124,0.18127,0.18131,0.18134,0.18138,0.18141,0.18145,0.18148,0.18152,0.18155,0.18159,0.18162,0.18166,0.18169,0.18173,0.18176,0.18179,0.18183;
      | 0.16551,0.16556,0.1656,0.16564,0.16569,0.16573,0.16577,0.16582,0.16586,0.1659,0.16594,0.16599,0.16603,0.16607,0.16612,0.16616,0.1662,0.16624,0.16629,0.16633,0.16637,0.16642,0.16646,0.1665,0.16654,0.16659,0.16663,0.16667,0.16671,0.16676,0.1668,0.16684,0.16688,0.16693,0.16697,0.16701,0.16705,0.1671,0.16714,0.16718,0.16722,0.16727,0.16731,0.16735,0.16739,0.16743,0.16748,0.16752,0.16756,0.1676,0.16764,0.16769,0.16773,0.16777,0.16781,0.16785,0.1679,0.16794,0.16798,0.16802;
      | 0.0080721,0.15115,0.1512,0.15125,0.1513,0.15136,0.15141,0.15146,0.15151,0.15156,0.15162,0.15167,0.15172,0.15177,0.15182,0.15187,0.15193,0.15198,0.15203,0.15208,0.15213,0.15218,0.15223,0.15228,0.15234,0.15239,0.15244,0.15249,0.15254,0.15259,0.15264,0.15269,0.15274,0.1528,0.15285,0.1529,0.15295,0.153,0.15305,0.1531,0.15315,0.1532,0.15325,0.1533,0.15335,0.1534,0.15345,0.15351,0.15356,0.15361,0.15366,0.15371,0.15376,0.15381,0.15386,0.15391,0.15396,0.15401,0.15406,0.15411;
      | 0.0090396,0.0091429,0.0092543,0.13659,0.13665,0.13671,0.13677,0.13684,0.1369,0.13696,0.13702,0.13709,0.13715,0.13721,0.13727,0.13733,0.1374,0.13746,0.13752,0.13758,0.13764,0.13771,0.13777,0.13783,0.13789,0.13795,0.13801,0.13807,0.13814,0.1382,0.13826,0.13832,0.13838,0.13844,0.1385,0.13856,0.13862,0.13868,0.13875,0.13881,0.13887,0.13893,0.13899,0.13905,0.13911,0.13917,0.13923,0.13929,0.13935,0.13941,0.13947,0.13953,0.13959,0.13965,0.13971,0.13977,0.13983,0.13989,0.13995,0.14001;
      | 0.01,0.010091,0.010187,0.010288,0.010395,0.010509,0.010632,0.12192,0.122,0.12208,0.12215,0.12223,0.1223,0.12238,0.12245,0.12253,0.1226,0.12268,0.12275,0.12283,0.1229,0.12298,0.12305,0.12312,0.1232,0.12327,0.12335,0.12342,0.12349,0.12357,0.12364,0.12371,0.12379,0.12386,0.12393,0.12401,0.12408,0.12415,0.12422,0.1243,0.12437,0.12444,0.12451,0.12459,0.12466,0.12473,0.1248,0.12487,0.12495,0.12502,0.12509,0.12516,0.12523,0.1253,0.12537,0.12545,0.12552,0.12559,0.12566,0.12573;
      | 0.010953,0.011035,0.011119,0.011207,0.011299,0.011395,0.011495,0.0116,0.01171,0.011826,0.011949,0.01208,0.012221,0.012373,0.10725,0.10734,0.10743,0.10753,0.10762,0.10771,0.1078,0.1079,0.10799,0.10808,0.10817,0.10826,0.10836,0.10845,0.10854,0.10863,0.10872,0.10881,0.1089,0.10899,0.10908,0.10917,0.10926,0.10935,0.10944,0.10953,0.10962,0.1097,0.10979,0.10988,0.10997,0.11006,0.11015,0.11023,0.11032,0.11041,0.1105,0.11058,0.11067,0.11076,0.11084,0.11093,0.11101,0.1111,0.11119,0.11127;
      | 0.011896,0.01197,0.012047,0.012126,0.012206,0.01229,0.012376,0.012465,0.012557,0.012653,0.012752,0.012855,0.012962,0.013074,0.013192,0.013315,0.013444,0.01358,0.013725,0.013878,0.014043,0.014219,0.01441,0.014619,0.014849,0.092711,0.092831,0.092951,0.09307,0.093189,0.093308,0.093426,0.093544,0.093661,0.093777,0.093894,0.09401,0.094125,0.09424,0.094355,0.094469,0.094583,0.094696,0.094809,0.094922,0.095034,0.095146,0.095257,0.095368,0.095479,0.09559,0.0957,0.095809,0.095919,0.096028,0.096136,0.096245,0.096353,0.09646,0.096568] W/(m*K)
  Lox Tank (Lox) : SimscapeFluids_lib/Thermal Liquid/Tanks & Accumulators/Tank (G-TL)  num_inlet=1  volume_total=19.88 l  volume_spec=fluids.thermal_liquid.tanks_accumulators.enum.TankVolumeSpec.Constant  tank_area=0.35 ft^2  level_TLU=[0, 3, 5] m  volume_TLU=[0, 4, 6] m^3  inlet_areas_A1B1=[1, 1] in^2  inlet_height_A2=0 in  inlet_area_A2=0.78 in^2  inlet_heights_A2B2=[.1, .1] m  inlet_areas_A2B2=[.01, .01] m^2  inlet_heights_A2B2C2=[.1, .1, .1] m  inlet_areas_A2B2C2=[.01, .01, .01] m^2  inlet_heights_A2B2C2D2=0.1 * ones(1, 4) m  inlet_areas_A2B2C2D2=0.01 * ones(1, 4) m^2  inlet_heights_A2B2C2D2E2=0.1 * ones(1, 5) m  inlet_areas_A2B2C2D2E2=0.01 * ones(1, 5) m^2  inlet_heights_A2B2C2D2E2F2=0.1 * ones(1, 6) m  inlet_areas_A2B2C2D2E2F2=0.01 * ones(1, 6) m^2  capacity_check=0  max_liquid_capacity=85 l  g=9.81 m/s^2  level_specify=off  level_priority=None  level=20.5 in  level_nominal_specify=off  level_nominal_value=1  level_nominal_unit=m  volume_liquid_specify=off  volume_liquid_priority=High  volume_liquid=16.9 l  volume_liquid_nominal_specify=off  volume_liquid_nominal_value=1  volume_liquid_nominal_unit=m^3  mass_liquid_specify=on  mass_liquid_priority=High  mass_liquid=19.43 kg  mass_liquid_nominal_specify=off  mass_liquid_nominal_value=1  mass_liquid_nominal_unit=kg  T_liquid_specify=on  T_liquid_priority=High  T_liquid=100 K  T_liquid_nominal_specify=off  T_liquid_nominal_value=1  T_liquid_nominal_unit=K  p_gas_specify=on  p_gas_priority=High  p_gas=500 psi  p_gas_nominal_specify=off  p_gas_nominal_value=1  p_gas_nominal_unit=MPa  T_gas_specify=off  T_gas_priority=Low  T_gas=150 K  T_gas_nominal_specify=off  T_gas_nominal_value=150  T_gas_nominal_unit=K  rho_gas_specify=off  rho_gas_priority=None  rho_gas=1.2 kg/m^3  rho_gas_nominal_specify=off  rho_gas_nominal_value=1  rho_gas_nominal_unit=kg/m^3
  Lox Temp : Scope  Commented=on
      settings: ActiveDisplayYMinimum=100.00021777589856  ActiveDisplayYMaximum=100.09752541003098  DataLoggingVariableName=ScopeData10
  Mass & Energy Flow Rate Sensor (TL)1 : fl_lib/Thermal Liquid/Sensors/Flow Rate Sensor (TL)  Commented=on  mass_flow_measure=true  volumetric_flow_measure=false  energy_flow_measure=true
  N2 Temp Lox Tank : Scope  Commented=on
      settings: ActiveDisplayYMinimum=266.22531987698528  ActiveDisplayYMaximum=300.41878389754385  DataLoggingVariableName=ScopeData12
  PS-Simulink Converter{1..4,6} (5 alike) : nesl_utility/PS-Simulink Converter  Commented=on  PhysicalDomain=network_engine_domain  SubClassName=ps_output  LeftPortType=input  RightPortType=output  PseudoPeriodic=off  Frequencies=[]  VectorFormat=inherit  Unit=inherit  AffineConversion=off
  Simulink-PS Converter2 : nesl_utility/Simulink-PS Converter  Commented=on  PhysicalDomain=network_engine_domain  SubClassName=ps_input  LeftPortType=input  RightPortType=output  PseudoPeriodic=off  Frequencies=[]  NoiseDistribution=none  NoiseParameters=[]  Unit=1  AffineConversion=off  FilteringAndDerivatives=provide  SimscapeFilterOrder=1  InputFilterTimeConstant=0.001  UdotUserProvided=0
  Sum : Sum  Commented=on  Inputs=|-+
  Switch3 : Switch  Commented=on  Criteria=u2 > Threshold  Threshold=155  SaturateOnIntegerOverflow=off  InputSameDT=off
  Temperature Sensor : fl_lib/Thermal/Thermal Sensors/Temperature Sensor  Commented=on  temperature_measure=foundation.enum.MeasurementReference.difference
  Temperature Sensor1 : fl_lib/Thermal/Thermal Sensors/Temperature Sensor  Commented=on  temperature_measure=foundation.enum.MeasurementReference.difference
  Thermal Ref (0K) : fl_lib/Thermal/Thermal Elements/Thermal Reference  Commented=on
  Thermal Ref (0K)1 : fl_lib/Thermal/Thermal Elements/Thermal Reference  Commented=on
  Thermal Ref2 (0K) : fl_lib/Thermal/Thermal Elements/Thermal Reference  Commented=on
  Conn1 : PMIOPort  Side=Right
  Conn3 : PMIOPort  Port=2  Side=Left
  wires:
  Switch3/1 -> Simulink-PS Converter2/1
  PS-Simulink Converter4/1 -> Switch3/2
  Constant2/1 -> Switch3/1
  Constant3/1 -> Switch3/3
  Constant/1 -> Sum/2
  Integrator/1 -> Sum/1
  Sum/1 -> Lox Mass Rate/1
  PS-Simulink Converter6/1 -> Lox Mass Flow Rate/1, Integrator/1
  PS-Simulink Converter2/1 -> Lox Temp/1
  PS-Simulink Converter3/1 -> N2 Temp Lox Tank/1
  PS-Simulink Converter1/1 -> Lox Liquid Level/1
  connections:
  Lox CdA/RConn1 -- Conn1/RConn1
  Simulink-PS Converter2/RConn1 -- Controlled Heat Flow Rate Source/RConn1
  Thermal Ref (0K)1/LConn1 -- Controlled Heat Flow Rate Source/RConn2
  Lox Properties from NIST/RConn1 -- Lox CdA/LConn1 -- Lox Tank (Lox)/LConn3
  PS-Simulink Converter2/LConn1 -- Temperature Sensor/RConn2
  Lox Tank (Lox)/LConn5 -- PS-Simulink Converter1/LConn1
  Conn3/RConn1 -- Lox Tank (Lox)/LConn1
  Lox Tank (Lox)/RConn1 -- Controlled Heat Flow Rate Source/LConn1 -- Temperature Sensor1/LConn1
  Temperature Sensor1/RConn1 -- Thermal Ref2 (0K)/LConn1
  Temperature Sensor/RConn1 -- Thermal Ref (0K)/LConn1
  PS-Simulink Converter6/LConn1 -- Mass & Energy Flow Rate Sensor (TL)1/RConn2
  Temperature Sensor1/RConn2 -- PS-Simulink Converter4/LConn1 -- PS-Simulink Converter3/LConn1
  Temperature Sensor/LConn1 -- Lox Tank (Lox)/RConn2

== system hopper_6dof/Mass_Propulsion/Propulsion/Propulsion_Fluid_Network/Fluid_Network/MR Feedback Loop ==
  Actual MR : Inport
  Commanded MR : Inport  Port=2
  PID Controller : slpidlib/PID Controller  Controller=PID  Form=Parallel  TimeDomain=Continuous-time  UseExternalTs=off  SampleTime=-1  IntegratorMethod=Forward Euler  FilterMethod=Forward Euler  ControllerParametersSource=internal  P=0.1  I=1.0  UseKiTs=off  D=0.75  UseExternalDerivativeSource=off  N=20  UseFilter=on  TunerSelectOption=Transfer Function Based (PID Tuner App)  InitialConditionSource=internal  InitialConditionForIntegrator=0  InitialConditionForFilter=0  DifferentiatorICPrevScaledInput=0  ExternalReset=none  TrackingMode=off  Kt=1  LimitOutput=off  SatLimitsSource=internal  UpperSaturationLimit=inf  LowerSaturationLimit=-inf  LinearizeAsGain=on  AntiWindupMode=none  Kb=1  LimitIntegrator=off  UpperIntegratorSaturationLimit=inf  LowerIntegratorSaturationLimit=-inf  POutMin=[]  POutMax=[]  IOutMin=[]  IOutMax=[]  DOutMin=[]  DOutMax=[]  NOutMin=[]  NOutMax=[]  SumOutMin=[]  SumOutMax=[]  SaturationOutMin=[]  SaturationOutMax=[]  PParamMin=[]  PParamMax=[]  IParamMin=[]  IParamMax=[]  DParamMin=[]  DParamMax=[]  NParamMin=[]  NParamMax=[]  KbParamMin=[]  KbParamMax=[]  KtParamMin=[]  KtParamMax=[]  KbOutMin=[]  KbOutMax=[]  KtOutMin=[]  KtOutMax=[]  IntegratorOutMin=[]  IntegratorOutMax=[]  FilterOutMin=[]  FilterOutMax=[]  SumI1OutMin=[]  SumI1OutMax=[]  SumI2OutMin=[]  SumI2OutMax=[]  SumI3OutMin=[]  SumI3OutMax=[]  SumI4OutMin=[]  SumI4OutMax=[]  SumDOutMin=[]  SumDOutMax=[]  DifferentiatorOutMin=[]  DifferentiatorOutMax=[]  FilterDiffOutCoefMin=[]  FilterDiffOutCoefMax=[]  ReciprocalOutMin=[]  ReciprocalOutMax=[]  SumDenOutMin=[]  SumDenOutMax=[]  SumNumOutMin=[]  SumNumOutMax=[]  DivideOutMin=[]  DivideOutMax=[]  UdiffTsProdOutMin=[]  UdiffTsProdOutMax=[]  NTsProdOutMin=[]  NTsProdOutMax=[]  UintegralTsProdOutMin=[]  UintegralTsProdOutMax=[]  UngainTsProdOutMin=[]  UngainTsProdOutMax=[]  ClampingZeroOutDataTypeStr=Inherit: Inherit via back propagation  ClampingZeroOutMin=[]  ClampingZeroOutMax=[]  FilterDenConstantOutDataTypeStr=Inherit: Inherit via back propagation  FilterDenConstantOutMin=[]  FilterDenConstantOutMax=[]  PCopyOutDataTypeStr=Inherit: Inherit via back propagation  PCopyOutMin=[]  PCopyOutMax=[]  NCopyOutDataTypeStr=Inherit: Inherit via back propagation  NCopyOutMin=[]  NCopyOutMax=[]  IntegratorContinuousStateAttributes=''  IntegratorStateMustResolveToSignalObject=off  IntegratorRTWStateStorageClass=Auto  FilterContinuousStateAttributes=''  FilterStateMustResolveToSignalObject=off  FilterRTWStateStorageClass=Auto  ParallelPVariant=InternalParameters  IdealPVariant=Disabled  IVariant=InternalParameters  DVariant=InternalParameters  IntegratorVariant=Continuous  SatVariant=Disabled  AWVariant=Passthrough  PCopyVariant=Disabled  TRVariant=Disabled  FdbkBlocksVariant=Forward  IdealPFdbkVariant=Disabled  SatFdbkVariant=Disabled  DerivativeFilterVariant=ContFilter  NVariant=InternalParameters  NCopyVariant=Disabled  FilterICVariant=InternalICsFilter  IntegratorICVariant=InternalICs  ExternalResetVariant=Disabled  TRSumVariant=Passthrough  SumFdbkVariant=Disabled  SumVariant=Sum_PID  TsampFilterVariant=InternalTs  TsampNgainVariant=Passthrough  TsampIntegralVariant=Disabled_SignalSpec  ExternalSaturationOutDataTypeStr=Inherit: Same as second input  DerivativeSourceVariant=ErrorSignal  PreIntVariant=InternalPreInt
  Scope : Scope
      settings: ActiveDisplayYMinimum=-8.8083106676181941  ActiveDisplayYMaximum=16.933498382637875  DataLoggingVariableName=ScopeData41
  Sum : Sum  Inputs=|+-
  Transfer Fcn : TransferFcn  Denominator=[0.1 1]
  Gain : Outport
  wires:
  Commanded MR/1 -> Sum/1
  Actual MR/1 -> Transfer Fcn/1
  Transfer Fcn/1 -> Sum/2
  PID Controller/1 -> Gain/1, Scope/1
  Sum/1 -> PID Controller/1

== system hopper_6dof/Mass_Propulsion/Propulsion/Propulsion_Fluid_Network/Fluid_Network/Ox Tank PT + Initial Conditions ==
  Initial OT Pressure : InitialCondition  Value=500
  PS-Simulink Converter3 : nesl_utility/PS-Simulink Converter  PhysicalDomain=network_engine_domain  SubClassName=ps_output  LeftPortType=input  RightPortType=output  PseudoPeriodic=off  Frequencies=[]  VectorFormat=inherit  Unit=inherit  AffineConversion=off
  Pa to psi : Gain  Gain=0.000145038
  Pressure & Temperature Sensor (TL) : fl_lib/Thermal Liquid/Sensors/Pressure & Temperature Sensor (TL)  reference=foundation.enum.MeasurementReference.absolute  pressure=true  pressure_spec=foundation.enum.PressureMeasementSpec.Gauge  temperature=false
  Conn1 : PMIOPort  Side=Left
  Pup : Outport
  wires:
  PS-Simulink Converter3/1 -> Pa to psi/1
  Pa to psi/1 -> Initial OT Pressure/1
  Initial OT Pressure/1 -> Pup/1
  connections:
  Pressure & Temperature Sensor (TL)/LConn1 -- Conn1/RConn1
  PS-Simulink Converter3/LConn1 -- Pressure & Temperature Sensor (TL)/RConn1

== system hopper_6dof/Mass_Propulsion/Propulsion/Propulsion_Fluid_Network/Fluid_Network/Ox Tank PT + Initial Conditions1 ==
  Initial OT Pressure : InitialCondition  Value=500
  PS-Simulink Converter3 : nesl_utility/PS-Simulink Converter  PhysicalDomain=network_engine_domain  SubClassName=ps_output  LeftPortType=input  RightPortType=output  PseudoPeriodic=off  Frequencies=[]  VectorFormat=inherit  Unit=inherit  AffineConversion=off
  Pa to psi : Gain  Gain=0.000145038
  Pressure & Temperature Sensor (TL) : fl_lib/Thermal Liquid/Sensors/Pressure & Temperature Sensor (TL)  reference=foundation.enum.MeasurementReference.absolute  pressure=true  pressure_spec=foundation.enum.PressureMeasementSpec.Gauge  temperature=false
  Conn1 : PMIOPort  Side=Left
  Out1 : Outport
  wires:
  PS-Simulink Converter3/1 -> Pa to psi/1
  Pa to psi/1 -> Initial OT Pressure/1
  Initial OT Pressure/1 -> Out1/1
  connections:
  Pressure & Temperature Sensor (TL)/LConn1 -- Conn1/RConn1
  PS-Simulink Converter3/LConn1 -- Pressure & Temperature Sensor (TL)/RConn1

== system hopper_6dof/Mass_Propulsion/Propulsion/Propulsion_Fluid_Network/Fluid_Network/Ox Tank PT + Initial Conditions2 ==
  Initial OT Pressure : InitialCondition  Value=500
  PS-Simulink Converter3 : nesl_utility/PS-Simulink Converter  PhysicalDomain=network_engine_domain  SubClassName=ps_output  LeftPortType=input  RightPortType=output  PseudoPeriodic=off  Frequencies=[]  VectorFormat=inherit  Unit=inherit  AffineConversion=off
  Pa to psi : Gain  Gain=0.000145038
  Pressure & Temperature Sensor (TL) : fl_lib/Thermal Liquid/Sensors/Pressure & Temperature Sensor (TL)  reference=foundation.enum.MeasurementReference.absolute  pressure=true  pressure_spec=foundation.enum.PressureMeasementSpec.Gauge  temperature=false
  fuel line : PMIOPort  Side=Left
  Out1 : Outport
  wires:
  PS-Simulink Converter3/1 -> Pa to psi/1
  Pa to psi/1 -> Initial OT Pressure/1
  Initial OT Pressure/1 -> Out1/1
  connections:
  Pressure & Temperature Sensor (TL)/LConn1 -- fuel line/RConn1
  PS-Simulink Converter3/LConn1 -- Pressure & Temperature Sensor (TL)/RConn1

== system hopper_6dof/Mass_Propulsion/Propulsion/Propulsion_Fluid_Network/Fluid_Network/Physical Combustion Chamber1 ==
  pc : Inport
  Controlled Reservoir (TL) : fl_lib/Thermal Liquid/Elements/Reservoir (TL)  pressure_input=false  pressure_spec=foundation.enum.pressure_spec.atmospheric  reservoir_pressure=0.101325 MPa  temperature_input=true  reservoir_temperature=293.15 K  area=0.01 m^2  input_error_spec=foundation.enum.input_range_error.warn
  Controlled Reservoir (TL)1 : fl_lib/Thermal Liquid/Elements/Reservoir (TL)  pressure_input=false  pressure_spec=foundation.enum.pressure_spec.atmospheric  reservoir_pressure=0.101325 MPa  temperature_input=true  reservoir_temperature=293.15 K  area=0.01 m^2  input_error_spec=foundation.enum.input_range_error.warn
  Ox Tank PT + Initial Conditions2 : Subsystem
  PS Constant : fl_lib/Physical Signals/Sources/PS Constant  constant=293.15 K
  PS Constant1 : fl_lib/Physical Signals/Sources/PS Constant  constant=100 K
  Pressure Source (TL) : fl_lib/Thermal Liquid/Sources/Pressure Source (TL)  source_type=foundation.enum.constant_controlled.controlled  pressure_differential=0 MPa  power_spec=foundation.enum.power_spec.isentropic  area=0.01 m^2
  Pressure Source (TL)1 : fl_lib/Thermal Liquid/Sources/Pressure Source (TL)  source_type=foundation.enum.constant_controlled.controlled  pressure_differential=0 MPa  power_spec=foundation.enum.power_spec.isentropic  area=0.01 m^2
  Pressure Source (TL)2 : fl_lib/Thermal Liquid/Sources/Pressure Source (TL)  source_type=foundation.enum.constant_controlled.controlled  pressure_differential=0 MPa  power_spec=foundation.enum.power_spec.isentropic  area=0.01 m^2
  Scope11 : Scope
      settings: ActiveDisplayYMinimum=-62.499971643181354  ActiveDisplayYMaximum=562.49999684924239  DataLoggingVariableName=ScopeData48
  Simulink-PS Converter1 : nesl_utility/Simulink-PS Converter  PhysicalDomain=network_engine_domain  SubClassName=ps_input  LeftPortType=input  RightPortType=output  PseudoPeriodic=off  Frequencies=[]  NoiseDistribution=none  NoiseParameters=[]  Unit=1  AffineConversion=off  FilteringAndDerivatives=filter  SimscapeFilterOrder=1  InputFilterTimeConstant=0.001  UdotUserProvided=0
  Simulink-PS Converter2 : nesl_utility/Simulink-PS Converter  PhysicalDomain=network_engine_domain  SubClassName=ps_input  LeftPortType=input  RightPortType=output  PseudoPeriodic=off  Frequencies=[]  NoiseDistribution=none  NoiseParameters=[]  Unit=1  AffineConversion=off  FilteringAndDerivatives=filter  SimscapeFilterOrder=1  InputFilterTimeConstant=0.001  UdotUserProvided=0
  Simulink-PS Converter4 : nesl_utility/Simulink-PS Converter  PhysicalDomain=network_engine_domain  SubClassName=ps_input  LeftPortType=input  RightPortType=output  PseudoPeriodic=off  Frequencies=[]  NoiseDistribution=none  NoiseParameters=[]  Unit=1  AffineConversion=off  FilteringAndDerivatives=filter  SimscapeFilterOrder=1  InputFilterTimeConstant=0.001  UdotUserProvided=0
  fuel line : PMIOPort  Side=Right
  ox line : PMIOPort  Port=2  Side=Right
  wires:
  Ox Tank PT + Initial Conditions2/1(Out1) -> Scope11/1
  pc/1 -> Simulink-PS Converter4/1, Simulink-PS Converter2/1, Simulink-PS Converter1/1
  connections:
  Ox Tank PT + Initial Conditions2/LConn1 -- Pressure Source (TL)2/RConn1
  Simulink-PS Converter2/RConn1 -- Pressure Source (TL)2/LConn2
  Pressure Source (TL)1/LConn1 -- Controlled Reservoir (TL)/LConn1
  Pressure Source (TL)1/RConn1 -- ox line/RConn1
  fuel line/RConn1 -- Pressure Source (TL)/RConn1
  Pressure Source (TL)/LConn1 -- Pressure Source (TL)2/LConn1 -- Controlled Reservoir (TL)1/LConn1
  Simulink-PS Converter1/RConn1 -- Pressure Source (TL)1/LConn2
  Simulink-PS Converter4/RConn1 -- Pressure Source (TL)/LConn2
  Controlled Reservoir (TL)1/RConn1 -- PS Constant/RConn1
  PS Constant1/RConn1 -- Controlled Reservoir (TL)/RConn1
